simulink model "inductionmotor_drive"  (R2023a)
settings: Solver=VariableStepAuto  StartTime=0.0  StopTime=5  RelTol=1e-3
libraries: spsMosfetLib x6, simulink x1, spsAsynchronousMachinepuUnitsLib x1, spsDCVoltageSourceLib x1, slpidlib x1, spsSawtoothGeneratorLib x1, spsThreePhaseVIMeasurementLib x1, sps_lib x1
settings Model: Creator=singh  LastModifiedBy=singh
settings DebuggingCC: ParameterPrecisionLossMsg=none

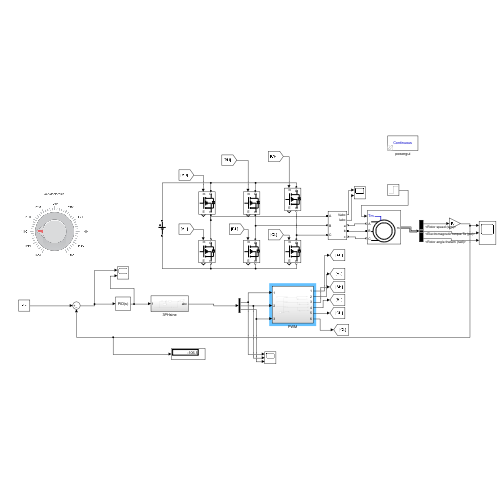
[thumbnail: Simulink's stored preview of the top-level diagram]
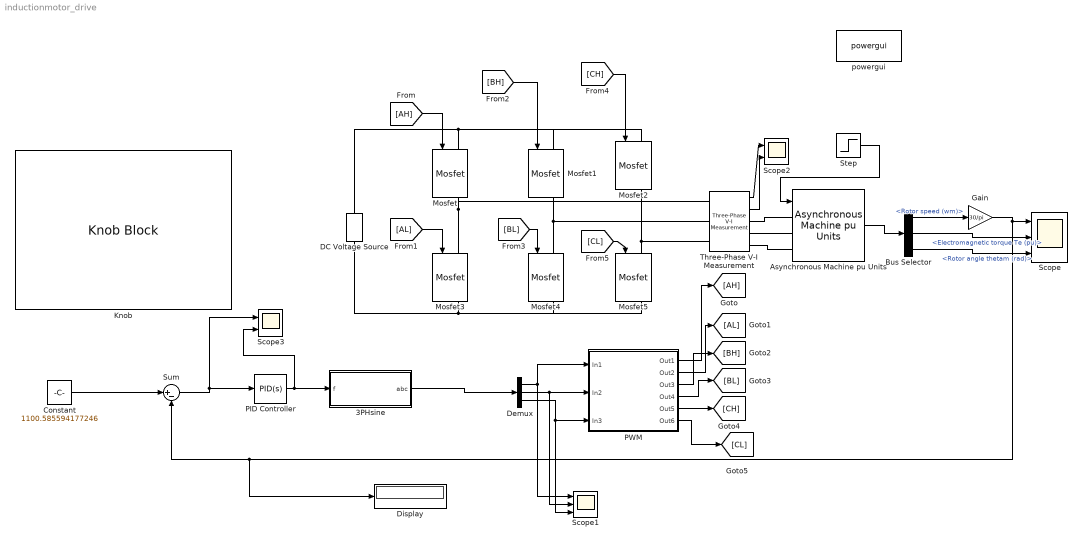
== system inductionmotor_drive ==
  3PHsine : Subsystem
  Asynchronous Machine pu Units : spsAsynchronousMachinepuUnitsLib/Asynchronous Machine pu Units  RotorType=Squirrel-cage  PresetModel="01:  5 HP   460 V 60Hz 1750 RPM"  MechanicalLoad=Torque Tm  ShowDetailedParameters=on  ReferenceFrame=Rotor  Units=pu  MeasurementBus=off  NominalParameters=[3730 460 60]  VoltageRatio=1  Stator=[0.01965 0.0397]  Rotor=[0.01909 0.0397]  Cage1=[0.01909 0.0397]  Cage2=[0.01909 0.0397]  Lm=1.354  Mechanical=[0.09526 0.05479 2]  PolePairs=2  InitialConditions="[ 1,0   0,0,0   0,0,0 ]"  SimulateSaturation=off  Saturation="[0.212,0.4201,0.8125,1.0979,1.4799,2.2457,3.2586,4.5763,6.4763 ;   0.5,0.7,0.9,1,1.1,1.2 ,1.3,1.4,1.5]"  LoadFlowParameters=0  TsPowergui=0  TsBlock=-1  IterativeModel=Trapezoidal non iterative  IterativeDiscreteModel=Trapezoidal non iterative  Pmec=0
      settings: LibrarySourceBlock=|
      | sps_lib/Electrical Machines/Asynchronous Machine
      | pu Units
  Bus Selector : BusSelector  OutputSignals=Mechanical.Rotor speed (wm),Mechanical.Electromagnetic torque Te (pu),Mechanical.Rotor angle thetam (rad)
  Constant : Constant  Value=1100.585594177246  OutMin=1000  OutMax=1500
  DC Voltage Source : spsDCVoltageSourceLib/DC Voltage Source  Amplitude=600  Measurements=None
  Demux : Demux  Outputs=3
  Display : Display
  Gain : Gain  Gain=30/pi
  Knob : KnobBlock  ScaleMin=1000  ScaleMax=1500
  Mosfet{,1..5} (6 alike) : spsMosfetLib/Mosfet  Ron=0.1  Lon=0  Rd=0.01  Vfd=0  IC=0  Rs=1e5  Cs=inf  Measurements=on
  PID Controller : slpidlib/PID Controller  Controller=PID  Form=Parallel  TimeDomain=Continuous-time  UseExternalTs=off  SampleTime=-1  IntegratorMethod=Forward Euler  FilterMethod=Forward Euler  ControllerParametersSource=internal  P=0.01  I=0.1  UseKiTs=off  D=0  N=100  UseFilter=on  TunerSelectOption=Transfer Function Based (PID Tuner App)  InitialConditionSource=internal  InitialConditionForIntegrator=0  InitialConditionForFilter=0  DifferentiatorICPrevScaledInput=0  ExternalReset=none  TrackingMode=off  Kt=1  LimitOutput=off  SatLimitsSource=internal  UpperSaturationLimit=inf  LowerSaturationLimit=-inf  LinearizeAsGain=on  AntiWindupMode=none  Kb=1  LimitIntegrator=off  UpperIntegratorSaturationLimit=inf  LowerIntegratorSaturationLimit=-inf  POutMin=[]  POutMax=[]  IOutMin=[]  IOutMax=[]  DOutMin=[]  DOutMax=[]  NOutMin=[]  NOutMax=[]  SumOutMin=[]  SumOutMax=[]  SaturationOutMin=[]  SaturationOutMax=[]  PParamMin=[]  PParamMax=[]  IParamMin=[]  IParamMax=[]  DParamMin=[]  DParamMax=[]  NParamMin=[]  NParamMax=[]  KbParamMin=[]  KbParamMax=[]  KtParamMin=[]  KtParamMax=[]  KbOutMin=[]  KbOutMax=[]  KtOutMin=[]  KtOutMax=[]  IntegratorOutMin=[]  IntegratorOutMax=[]  FilterOutMin=[]  FilterOutMax=[]  SumI1OutMin=[]  SumI1OutMax=[]  SumI2OutMin=[]  SumI2OutMax=[]  SumI3OutMin=[]  SumI3OutMax=[]  SumI4OutMin=[]  SumI4OutMax=[]  SumDOutMin=[]  SumDOutMax=[]  DifferentiatorOutMin=[]  DifferentiatorOutMax=[]  FilterDiffOutCoefMin=[]  FilterDiffOutCoefMax=[]  ReciprocalOutMin=[]  ReciprocalOutMax=[]  SumDenOutMin=[]  SumDenOutMax=[]  SumNumOutMin=[]  SumNumOutMax=[]  DivideOutMin=[]  DivideOutMax=[]  UdiffTsProdOutMin=[]  UdiffTsProdOutMax=[]  NTsProdOutMin=[]  NTsProdOutMax=[]  UintegralTsProdOutMin=[]  UintegralTsProdOutMax=[]  UngainTsProdOutMin=[]  UngainTsProdOutMax=[]  ClampingZeroOutDataTypeStr=Inherit: Inherit via back propagation  ClampingZeroOutMin=[]  ClampingZeroOutMax=[]  FilterDenConstantOutDataTypeStr=Inherit: Inherit via back propagation  FilterDenConstantOutMin=[]  FilterDenConstantOutMax=[]  PCopyOutDataTypeStr=Inherit: Inherit via back propagation  PCopyOutMin=[]  PCopyOutMax=[]  NCopyOutDataTypeStr=Inherit: Inherit via back propagation  NCopyOutMin=[]  NCopyOutMax=[]  IntegratorContinuousStateAttributes=''  IntegratorStateMustResolveToSignalObject=off  IntegratorRTWStateStorageClass=Auto  FilterContinuousStateAttributes=''  FilterStateMustResolveToSignalObject=off  FilterRTWStateStorageClass=Auto  ParallelPVariant=InternalParameters  IdealPVariant=Disabled  IVariant=InternalParameters  DVariant=InternalParameters  IntegratorVariant=Continuous  SatVariant=Disabled  AWVariant=Passthrough  PCopyVariant=Disabled  TRVariant=Disabled  FdbkBlocksVariant=Forward  IdealPFdbkVariant=Disabled  SatFdbkVariant=Disabled  DerivativeFilterVariant=ContFilter  NVariant=InternalParameters  NCopyVariant=Disabled  FilterICVariant=InternalICsFilter  IntegratorICVariant=InternalICs  ExternalResetVariant=Disabled  TRSumVariant=Passthrough  SumFdbkVariant=Disabled  SumVariant=Sum_PID  TsampFilterVariant=InternalTs  TsampNgainVariant=Passthrough  TsampIntegralVariant=Disabled_SignalSpec  ExternalSaturationOutDataTypeStr=Inherit: Same as second input
  PWM : Subsystem
  Scope : Scope  NumInputPorts=3
  Scope1 : Scope  NumInputPorts=3
  Scope2 : Scope  NumInputPorts=2
  Scope3 : Scope  NumInputPorts=2
  Step : Step  SampleTime=0
  Sum : Sum  Inputs=|+-
  Three-Phase V-I Measurement : spsThreePhaseVIMeasurementLib/Three-Phase V-I Measurement  VoltageMeasurement=phase-to-phase  SetLabelV=off  LabelV=Vabc  Vpu=off  VpuLL=off  CurrentMeasurement=yes  SetLabelI=off  LabelI=Iabc  Ipu=off  Pbase=100e6  Vbase=500e3  OutputType=Complex  PhasorSimulation=off  PSBequivalent=0
  powergui : sps_lib/powergui  Priority=1  SimulationMode=Continuous  SampleTime=50e-6  frequency=60  Iterations=50  frequencyindice=0  Pbase=100e6  ErrMax=1e-4  UnitsV=kV  UnitsW=MW  buscounter=0  FunctionMessages=off  echomessages=off  EnableUseOfTLC=off  CurrentSourceSwitches=off  DisableSnubberDevices=off  DisableRonSwitches=off  DisableVfSwitches=off  DisplayEquations=off  AutomaticDiscreteSolvers=off  SolverType=Tustin/Backward Euler (TBE)  Interpol=off  ExternalGateDelay=off  methode=off  Ts=100  x0status=blocks  SPID=on  SwTol=0  HookPort=off  NonlinearTolerance=1e-4  nMaxIteration=100  ContinueOnMaxIteration=off  RestoreLinks=warning  ResistiveCurrentMeasurement=off  Frange=[0:2:500]  Ylog=off  Xlog=on  ShowGrid=off  save=off  variable=ZData  structure=0  ZoomFFT=off  StartTime=0.0  cycles=1  DisplayStyle=1  fundamental=60  FreqAxis=off  MaxFrequency=1000  frequencyindicesteady=1  RmsSteady=1  display=off
  wires:
  Bus Selector/1 -> Gain/1  "<Rotor speed (wm)>"
  Gain/1 -> Display/1, Sum/2, Scope/1
  Bus Selector/2 -> Scope/2  "<Electromagnetic torque Te (pu)>"
  Bus Selector/3 -> Scope/3  "<Rotor angle thetam (rad)>"
  Constant/1 -> Sum/1
  Sum/1 -> PID Controller/1, Scope3/1
  PID Controller/1 -> Scope3/2, 3PHsine/1(f)
  Demux/1 -> Scope1/1, PWM/1(In1)
  Demux/2 -> PWM/2(In2), Scope1/2
  Demux/3 -> PWM/3(In3), Scope1/3
  PWM/1(Out1) -> [AH]
  PWM/2(Out2) -> [AL]
  PWM/3(Out3) -> [BH]
  PWM/4(Out4) -> [BL]
  PWM/5(Out5) -> [CH]
  PWM/6(Out6) -> [CL]
  [AH] -> Mosfet/1
  [AL] -> Mosfet3/1
  [CL] -> Mosfet5/1
  [CH] -> Mosfet2/1
  [BH] -> Mosfet1/1
  [BL] -> Mosfet4/1
  Three-Phase V-I Measurement/1 -> Scope2/1
  Three-Phase V-I Measurement/2 -> Scope2/2
  Asynchronous Machine pu Units/1 -> Bus Selector/1
  Step/1 -> Asynchronous Machine pu Units/1
  3PHsine/1(abc) -> Demux/1
  connections:
  DC Voltage Source/RConn1 -- Mosfet2/LConn1 -- Mosfet1/LConn1 -- Mosfet/LConn1
  DC Voltage Source/LConn1 -- Mosfet5/RConn1 -- Mosfet4/RConn1 -- Mosfet3/RConn1
  Mosfet1/RConn1 -- Mosfet4/LConn1 -- Three-Phase V-I Measurement/LConn2
  Mosfet/RConn1 -- Mosfet3/LConn1 -- Three-Phase V-I Measurement/LConn1
  Mosfet2/RConn1 -- Three-Phase V-I Measurement/LConn3 -- Mosfet5/LConn1
  Asynchronous Machine pu Units/LConn1 -- Three-Phase V-I Measurement/RConn1
  Asynchronous Machine pu Units/LConn2 -- Three-Phase V-I Measurement/RConn2
  Asynchronous Machine pu Units/LConn3 -- Three-Phase V-I Measurement/RConn3

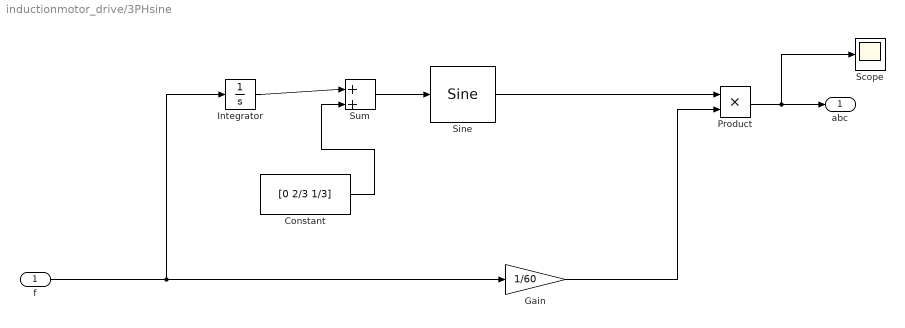
== system inductionmotor_drive/3PHsine ==
  f : Inport
  Constant : Constant  Value=[0 2/3 1/3]
  Gain : Gain  Gain=1/60
  Integrator : Integrator  IgnoreLimit=on
  Product : Product
  Scope : Scope
  Sine : simulink/Lookup Tables/Sine  Formula=sin(2*pi*u)  NumDataPoints=(2^5)+1  OutputWordLength=16  InternalRulePriority=Speed
  Sum : Sum  Inputs=|++
  abc : Outport
  wires:
  Integrator/1 -> Sum/1
  Sum/1 -> Sine/1
  Gain/1 -> Product/2
  f/1 -> Integrator/1, Gain/1
  Constant/1 -> Sum/2
  Product/1 -> Scope/1, abc/1
  Sine/1 -> Product/1

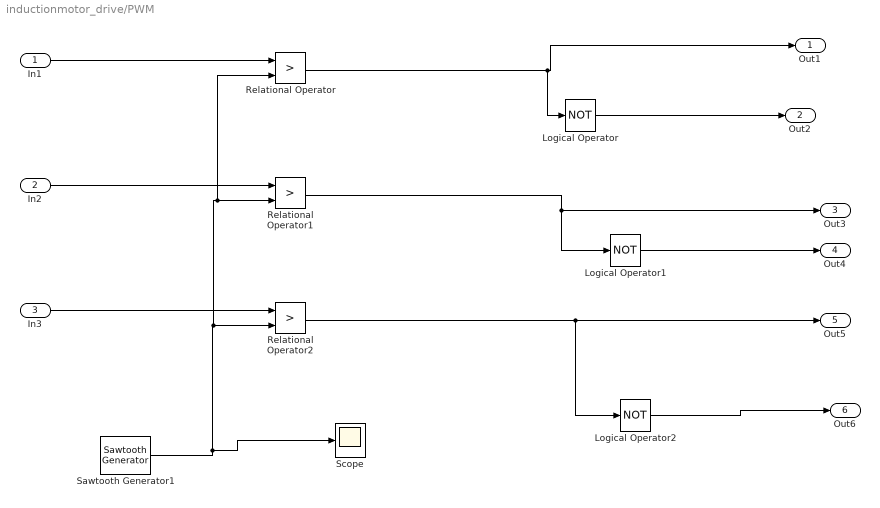
== system inductionmotor_drive/PWM ==
  In1 : Inport
  In2 : Inport  Port=2
  In3 : Inport  Port=3
  Logical Operator : Logic  Operator=NOT  IconShape=distinctive  AllPortsSameDT=off  OutDataTypeStr=boolean
  Logical Operator1 : Logic  Operator=NOT  IconShape=distinctive  AllPortsSameDT=off  OutDataTypeStr=boolean
  Logical Operator2 : Logic  Operator=NOT  IconShape=distinctive  AllPortsSameDT=off  OutDataTypeStr=boolean
  Relational Operator : RelationalOperator  Operator=>  OutDataTypeStr=boolean  RndMeth=Simplest  InputSameDT=off
  Relational Operator1 : RelationalOperator  Operator=>  OutDataTypeStr=boolean  RndMeth=Simplest  InputSameDT=off
  Relational Operator2 : RelationalOperator  Operator=>  OutDataTypeStr=boolean  RndMeth=Simplest  InputSameDT=off
  Sawtooth Generator1 : spsSawtoothGeneratorLib/Sawtooth Generator  Freq=1e3  Phase=180  Ts=0
  Scope : Scope
  Out1 : Outport
  Out2 : Outport  Port=2
  Out3 : Outport  Port=3
  Out4 : Outport  Port=4
  Out5 : Outport  Port=5
  Out6 : Outport  Port=6
  wires:
  In1/1 -> Relational Operator/1
  In3/1 -> Relational Operator2/1
  Logical Operator/1 -> Out2/1
  Relational Operator/1 -> Logical Operator/1, Out1/1
  Relational Operator1/1 -> Out3/1, Logical Operator1/1
  Logical Operator1/1 -> Out4/1
  Logical Operator2/1 -> Out6/1
  Relational Operator2/1 -> Logical Operator2/1, Out5/1
  Sawtooth Generator1/1 -> Relational Operator/2, Relational Operator1/2, Relational Operator2/2, Scope/1
  In2/1 -> Relational Operator1/1
